simulink model "FSI_1DOF_SS_TF_Simulink"  (R2018b)
settings: Solver=FixedStepAuto  StartTime=0.0  StopTime=5  FixedStep=1e-4  RelTol=1e-3  EnableMultiTasking=on
undefined symbols (not defined in the file): A1, B1, bias, C1, D1, den_1DOF, F, isel, num_1DOF, omega, phase, t_step, v_10, x_10
settings Model: Creator=FilipKsica  LastModifiedBy=FilipKsica
settings DataIOCC: LimitDataPoints=on
settings OptimizationCC: LifeSpan=inf
settings DebuggingCC: AllowSymbolicDim=off  SFUnexpectedBacktrackingDiag=warning  SFNoUnconditionalDefaultTransitionDiag=warning  SFExecutionAtInitializationDiag=none
settings ModelReferenceCC: PropagateSignalLabelsOutOfModel=off
settings SFSimCC: SimUseLocalCustomCode=off
settings RTWCC: RTWUseLocalCustomCode=off
settings CodeAppCC: StateflowObjectComments=on
settings GRTTargetCC: TargetLangStandard=C89/C90 (ANSI)
settings ConfigComp: CovMetricSettings=dw  CovHtmlReporting=on  CovSaveCumulativeToWorkspaceVar=on  CovSaveSingleToWorkspaceVar=on  CovExternalEMLEnable=off

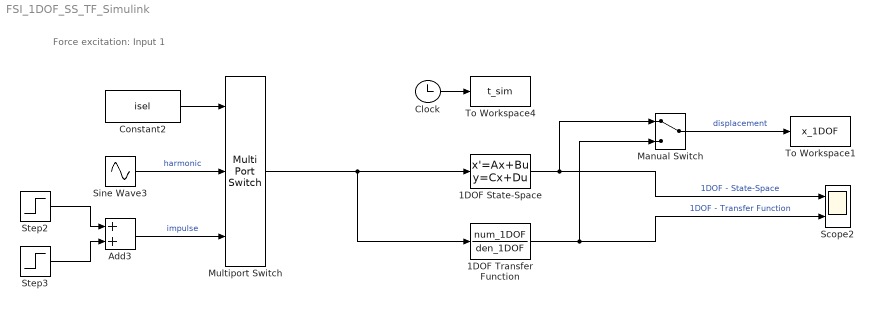
== system FSI_1DOF_SS_TF_Simulink ==
  note: Force excitation: Input 1
  1DOF State-Space : StateSpace  A=A1  B=B1  C=C1  D=D1  InitialCondition=[x_10 v_10]
  1DOF Transfer Function : TransferFcn  Numerator=num_1DOF  Denominator=den_1DOF
  Add3 : Sum
  Clock : Clock
  Constant2 : Constant  Value=isel
  Manual Switch : ManualSwitch
  Multiport Switch : MultiPortSwitch  Inputs=2
  Scope2 : Scope  NumInputPorts=2
  Sine Wave3 : Sin  Amplitude=F  Bias=bias  Frequency=omega  Phase=phase  SampleTime=0
  Step2 : Step  Time=0  After=F  SampleTime=0
  Step3 : Step  Time=t_step  After=-F  SampleTime=0
  To Workspace1 : ToWorkspace  VariableName=x_1DOF  SampleTime=-1
  To Workspace4 : ToWorkspace  VariableName=t_sim  SampleTime=-1
  wires:
  1DOF State-Space/1 -> Scope2/1, Manual Switch/1  "1DOF - State-Space"
  Clock/1 -> To Workspace4/1
  1DOF Transfer Function/1 -> Scope2/2, Manual Switch/2  "1DOF - Transfer Function"
  Manual Switch/1 -> To Workspace1/1  "displacement"
  Step3/1 -> Add3/2
  Sine Wave3/1 -> Multiport Switch/2  "harmonic"
  Add3/1 -> Multiport Switch/3  "impulse"
  Step2/1 -> Add3/1
  Constant2/1 -> Multiport Switch/1
  Multiport Switch/1 -> 1DOF Transfer Function/1, 1DOF State-Space/1
